simulink model "ASM_Traffic_MultiCore"  (R2026a)
settings: Solver=ode1  StartTime=SIM.tstart.v  StopTime=SIM.tend.v  FixedStep=SIM.StepSize.v
PostLoadFcn:
  | if any(exist('dsrtsu_mdlpostloadfcn', 'file') ~= 0), dsrtsu_mdlpostloadfcn('Execute', bdroot); end
  | try, asm_mdl_postloadfcn(bdroot, 'UpdateModel', 3600); catch, disp(lasterr); end,
InitFcn:
  | , if any(exist('rtifpga_mdlclblib', 'file') ~= 0), rtifpga_mdlclblib('Init', bdroot); end,
  | , if any(exist('dsmpb_private', 'file') ~= 0), dsmpb_private('dsmpb_mdlclblib', 'Init', bdroot); end,
model workspace (MAT data in the model file):
  asmReferencePath = [0 0.01 0.02 0.03 0.04 0.05 0.06 0.07 0.08 0.09 0.1 0.11 ... (350007 elements, 50001x7)]
  roadBounds : Simulink.Parameter (value not decoded)
  safetyAxes : Simulink.Parameter (value not decoded)
undefined symbols (not defined in the file): _to_, a0b2, ASM_BrakeHydraulics_DemoSystems, ASM_VehicleDynamics_DemoSystems, b98103fe8ad365046cd0, BrakeCircuit, controllerConfig, CPT, Crankshaft, DiscIntNeverNeededParam, dsmsi, FinalDriveAssembly, MDL, ModeSignals, mu, Pos_BrakePedal_Maneuver, rad, RefSignals, roadFamilyData, roadFamilyId, s_to_rpm, SIM, SoftECU, Suspension, Tire, Transmission
libraries: ASM_Traffic_lib x135, simulink x98, ASM_Utils_lib x77, ASM_VehicleDynamics_lib x70, ASM_Environment_lib x22, dsmpblib x20, dsmsilib x15, MDLD_Utils_lib x10, ASM_BrakeHydraulics_lib x3, sl_discontinuities x2
(part 55 of 65)

== system ASM_Traffic_MultiCore/VehicleDynamics/Plant/UserInterface/DISP_Plant/Positions/Angle_Pitch_Vehicle_CoorSys_E[deg] ==
  In1 : Inport
  Out1 : Outport  VectorParamsAs1DForOutWhenUnconnected=off
  wires:
  In1/1 -> Out1/1

== system ASM_Traffic_MultiCore/VehicleDynamics/Plant/UserInterface/DISP_Plant/Positions/Angle_Roll_Vehicle_CoorSys_E[deg] ==
  In1 : Inport
  Out1 : Outport  VectorParamsAs1DForOutWhenUnconnected=off
  wires:
  In1/1 -> Out1/1

== system ASM_Traffic_MultiCore/VehicleDynamics/Plant/UserInterface/DISP_Plant/Positions/Angle_Yaw_Vehicle_CoorSys_E[deg] ==
  In1 : Inport
  Out1 : Outport  VectorParamsAs1DForOutWhenUnconnected=off
  wires:
  In1/1 -> Out1/1

== system ASM_Traffic_MultiCore/VehicleDynamics/Plant/UserInterface/DISP_Plant/Positions/Pos_x_Vehicle_CoorSys_E[m] ==
  In1 : Inport
  Out1 : Outport  VectorParamsAs1DForOutWhenUnconnected=off
  wires:
  In1/1 -> Out1/1

== system ASM_Traffic_MultiCore/VehicleDynamics/Plant/UserInterface/DISP_Plant/Positions/Pos_y_Vehicle_CoorSys_E[m] ==
  In1 : Inport
  Out1 : Outport  VectorParamsAs1DForOutWhenUnconnected=off
  wires:
  In1/1 -> Out1/1

== system ASM_Traffic_MultiCore/VehicleDynamics/Plant/UserInterface/DISP_Plant/Positions/Pos_z_Vehicle_CoorSys_E[m] ==
  In1 : Inport
  Out1 : Outport  VectorParamsAs1DForOutWhenUnconnected=off
  wires:
  In1/1 -> Out1/1

== system ASM_Traffic_MultiCore/VehicleDynamics/Plant/UserInterface/DISP_Plant/Positions/s_Vehicle[m] ==
  In1 : Inport
  Out1 : Outport  VectorParamsAs1DForOutWhenUnconnected=off
  wires:
  In1/1 -> Out1/1

== system ASM_Traffic_MultiCore/VehicleDynamics/Plant/UserInterface/DISP_Plant/Sensor1/a_Angular_Sensor1_CoorSys_VH[x;y;z][rad|s2] ==
  In1 : Inport
  Out1 : Outport  VectorParamsAs1DForOutWhenUnconnected=off
  wires:
  In1/1 -> Out1/1

== system ASM_Traffic_MultiCore/VehicleDynamics/Plant/UserInterface/DISP_Plant/Sensor1/a_Angular_Sensor1_CoorSys_V[x;y;z][rad|s2] ==
  In1 : Inport
  Out1 : Outport  VectorParamsAs1DForOutWhenUnconnected=off
  wires:
  In1/1 -> Out1/1

== system ASM_Traffic_MultiCore/VehicleDynamics/Plant/UserInterface/DISP_Plant/Sensor1/a_Sensor1_CoorSys_VH[x;y;z][m|s2] ==
  In1 : Inport
  Out1 : Outport  VectorParamsAs1DForOutWhenUnconnected=off
  wires:
  In1/1 -> Out1/1

== system ASM_Traffic_MultiCore/VehicleDynamics/Plant/UserInterface/DISP_Plant/Sensor1/a_Sensor1_CoorSys_V[x;y;z][m|s2] ==
  In1 : Inport
  Out1 : Outport  VectorParamsAs1DForOutWhenUnconnected=off
  wires:
  In1/1 -> Out1/1

== system ASM_Traffic_MultiCore/VehicleDynamics/Plant/UserInterface/DISP_Plant/Sensor1/a_Total_Sensor1_CoorSys_VH[x;y;z][m|s2] ==
  In1 : Inport
  Out1 : Outport  VectorParamsAs1DForOutWhenUnconnected=off
  wires:
  In1/1 -> Out1/1

== system ASM_Traffic_MultiCore/VehicleDynamics/Plant/UserInterface/DISP_Plant/Sensor1/a_Total_Sensor1_CoorSys_V[x;y;z][m|s2] ==
  In1 : Inport
  Out1 : Outport  VectorParamsAs1DForOutWhenUnconnected=off
  wires:
  In1/1 -> Out1/1

== system ASM_Traffic_MultiCore/VehicleDynamics/Plant/UserInterface/DISP_Plant/Sensor1/v_Sensor1_CoorSys_VH[x;y;z][m|s] ==
  In1 : Inport
  Out1 : Outport  VectorParamsAs1DForOutWhenUnconnected=off
  wires:
  In1/1 -> Out1/1

== system ASM_Traffic_MultiCore/VehicleDynamics/Plant/UserInterface/DISP_Plant/Sensor1/v_Sensor1_CoorSys_V[x;y;z][m|s] ==
  In1 : Inport
  Out1 : Outport  VectorParamsAs1DForOutWhenUnconnected=off
  wires:
  In1/1 -> Out1/1

== system ASM_Traffic_MultiCore/VehicleDynamics/Plant/UserInterface/DISP_Plant/Sensor1/w_Sensor1_CoorSys_VH[x;y;z][rad|s] ==
  In1 : Inport
  Out1 : Outport  VectorParamsAs1DForOutWhenUnconnected=off
  wires:
  In1/1 -> Out1/1

== system ASM_Traffic_MultiCore/VehicleDynamics/Plant/UserInterface/DISP_Plant/Sensor1/w_Sensor1_CoorSys_V[x;y;z][rad|s] ==
  In1 : Inport
  Out1 : Outport  VectorParamsAs1DForOutWhenUnconnected=off
  wires:
  In1/1 -> Out1/1

== system ASM_Traffic_MultiCore/VehicleDynamics/Plant/UserInterface/DISP_Plant/Steering/Angle_SteeringGear[deg] ==
  In1 : Inport
  Out1 : Outport  VectorParamsAs1DForOutWhenUnconnected=off
  wires:
  In1/1 -> Out1/1

== system ASM_Traffic_MultiCore/VehicleDynamics/Plant/UserInterface/DISP_Plant/Steering/Angle_SteeringWheel[deg] ==
  In1 : Inport
  Out1 : Outport  VectorParamsAs1DForOutWhenUnconnected=off
  wires:
  In1/1 -> Out1/1

== system ASM_Traffic_MultiCore/VehicleDynamics/Plant/UserInterface/DISP_Plant/Steering/Displ_Steering[m] ==
  In1 : Inport
  Out1 : Outport  VectorParamsAs1DForOutWhenUnconnected=off
  wires:
  In1/1 -> Out1/1

== system ASM_Traffic_MultiCore/VehicleDynamics/Plant/UserInterface/DISP_Plant/Steering/Trq_PowerSteering[Nm] ==
  In1 : Inport
  Out1 : Outport  VectorParamsAs1DForOutWhenUnconnected=off
  wires:
  In1/1 -> Out1/1

== system ASM_Traffic_MultiCore/VehicleDynamics/Plant/UserInterface/DISP_Plant/Steering/Trq_Steering[Nm] ==
  In1 : Inport
  Out1 : Outport  VectorParamsAs1DForOutWhenUnconnected=off
  wires:
  In1/1 -> Out1/1

== system ASM_Traffic_MultiCore/VehicleDynamics/Plant/UserInterface/DISP_Plant/Steering/i_Steering_Mean[] ==
  In1 : Inport
  Out1 : Outport  VectorParamsAs1DForOutWhenUnconnected=off
  wires:
  In1/1 -> Out1/1

== system ASM_Traffic_MultiCore/VehicleDynamics/Plant/UserInterface/DISP_Plant/Suspension/Angle_Alpha_FL_Wheel[deg] ==
  In1 : Inport
  Out1 : Outport  VectorParamsAs1DForOutWhenUnconnected=off
  wires:
  In1/1 -> Out1/1

== system ASM_Traffic_MultiCore/VehicleDynamics/Plant/UserInterface/DISP_Plant/Suspension/Angle_Alpha_FR_Wheel[deg] ==
  In1 : Inport
  Out1 : Outport  VectorParamsAs1DForOutWhenUnconnected=off
  wires:
  In1/1 -> Out1/1

== system ASM_Traffic_MultiCore/VehicleDynamics/Plant/UserInterface/DISP_Plant/Suspension/Angle_Alpha_RL_Wheel[deg] ==
  In1 : Inport
  Out1 : Outport  VectorParamsAs1DForOutWhenUnconnected=off
  wires:
  In1/1 -> Out1/1

== system ASM_Traffic_MultiCore/VehicleDynamics/Plant/UserInterface/DISP_Plant/Suspension/Angle_Alpha_RR_Wheel[deg] ==
  In1 : Inport
  Out1 : Outport  VectorParamsAs1DForOutWhenUnconnected=off
  wires:
  In1/1 -> Out1/1

== system ASM_Traffic_MultiCore/VehicleDynamics/Plant/UserInterface/DISP_Plant/Suspension/Angle_Beta_FL_Wheel[deg] ==
  In1 : Inport
  Out1 : Outport  VectorParamsAs1DForOutWhenUnconnected=off
  wires:
  In1/1 -> Out1/1

== system ASM_Traffic_MultiCore/VehicleDynamics/Plant/UserInterface/DISP_Plant/Suspension/Angle_Beta_FR_Wheel[deg] ==
  In1 : Inport
  Out1 : Outport  VectorParamsAs1DForOutWhenUnconnected=off
  wires:
  In1/1 -> Out1/1

== system ASM_Traffic_MultiCore/VehicleDynamics/Plant/UserInterface/DISP_Plant/Suspension/Angle_Beta_RL_Wheel[deg] ==
  In1 : Inport
  Out1 : Outport  VectorParamsAs1DForOutWhenUnconnected=off
  wires:
  In1/1 -> Out1/1

== system ASM_Traffic_MultiCore/VehicleDynamics/Plant/UserInterface/DISP_Plant/Suspension/Angle_Beta_RR_Wheel[deg] ==
  In1 : Inport
  Out1 : Outport  VectorParamsAs1DForOutWhenUnconnected=off
  wires:
  In1/1 -> Out1/1

== system ASM_Traffic_MultiCore/VehicleDynamics/Plant/UserInterface/DISP_Plant/Suspension/Angle_FL_Wheel[Alpha;Beta;Gamma][deg] ==
  In1 : Inport
  Out1 : Outport  VectorParamsAs1DForOutWhenUnconnected=off
  wires:
  In1/1 -> Out1/1

== system ASM_Traffic_MultiCore/VehicleDynamics/Plant/UserInterface/DISP_Plant/Suspension/Angle_FRWheel[Alpha;Beta;Gamma][deg] ==
  In1 : Inport
  Out1 : Outport  VectorParamsAs1DForOutWhenUnconnected=off
  wires:
  In1/1 -> Out1/1

== system ASM_Traffic_MultiCore/VehicleDynamics/Plant/UserInterface/DISP_Plant/Suspension/Angle_Gamma_FL_Wheel[deg] ==
  In1 : Inport
  Out1 : Outport  VectorParamsAs1DForOutWhenUnconnected=off
  wires:
  In1/1 -> Out1/1

== system ASM_Traffic_MultiCore/VehicleDynamics/Plant/UserInterface/DISP_Plant/Suspension/Angle_Gamma_FR_Wheel[deg] ==
  In1 : Inport
  Out1 : Outport  VectorParamsAs1DForOutWhenUnconnected=off
  wires:
  In1/1 -> Out1/1

== system ASM_Traffic_MultiCore/VehicleDynamics/Plant/UserInterface/DISP_Plant/Suspension/Angle_Gamma_RL_Wheel[deg] ==
  In1 : Inport
  Out1 : Outport  VectorParamsAs1DForOutWhenUnconnected=off
  wires:
  In1/1 -> Out1/1

== system ASM_Traffic_MultiCore/VehicleDynamics/Plant/UserInterface/DISP_Plant/Suspension/Angle_Gamma_RR_Wheel[deg] ==
  In1 : Inport
  Out1 : Outport  VectorParamsAs1DForOutWhenUnconnected=off
  wires:
  In1/1 -> Out1/1

== system ASM_Traffic_MultiCore/VehicleDynamics/Plant/UserInterface/DISP_Plant/Suspension/Angle_RL_Wheel[Alpha;Beta;Gamma][deg] ==
  In1 : Inport
  Out1 : Outport  VectorParamsAs1DForOutWhenUnconnected=off
  wires:
  In1/1 -> Out1/1

== system ASM_Traffic_MultiCore/VehicleDynamics/Plant/UserInterface/DISP_Plant/Suspension/Angle_RR_Wheel[Alpha;Beta;Gamma][deg] ==
  In1 : Inport
  Out1 : Outport  VectorParamsAs1DForOutWhenUnconnected=off
  wires:
  In1/1 -> Out1/1

== system ASM_Traffic_MultiCore/VehicleDynamics/Plant/UserInterface/DISP_Plant/Suspension/Displ_Damper_FL[m] ==
  In1 : Inport
  Out1 : Outport  VectorParamsAs1DForOutWhenUnconnected=off
  wires:
  In1/1 -> Out1/1

== system ASM_Traffic_MultiCore/VehicleDynamics/Plant/UserInterface/DISP_Plant/Suspension/Displ_Damper_FL_dt[m|s] ==
  In1 : Inport
  Out1 : Outport  VectorParamsAs1DForOutWhenUnconnected=off
  wires:
  In1/1 -> Out1/1

== system ASM_Traffic_MultiCore/VehicleDynamics/Plant/UserInterface/DISP_Plant/Suspension/Displ_Damper_FR[m] ==
  In1 : Inport
  Out1 : Outport  VectorParamsAs1DForOutWhenUnconnected=off
  wires:
  In1/1 -> Out1/1

== system ASM_Traffic_MultiCore/VehicleDynamics/Plant/UserInterface/DISP_Plant/Suspension/Displ_Damper_FR_dt[m|s] ==
  In1 : Inport
  Out1 : Outport  VectorParamsAs1DForOutWhenUnconnected=off
  wires:
  In1/1 -> Out1/1

== system ASM_Traffic_MultiCore/VehicleDynamics/Plant/UserInterface/DISP_Plant/Suspension/Displ_Damper_RL[m] ==
  In1 : Inport
  Out1 : Outport  VectorParamsAs1DForOutWhenUnconnected=off
  wires:
  In1/1 -> Out1/1

== system ASM_Traffic_MultiCore/VehicleDynamics/Plant/UserInterface/DISP_Plant/Suspension/Displ_Damper_RL_dt[m|s] ==
  In1 : Inport
  Out1 : Outport  VectorParamsAs1DForOutWhenUnconnected=off
  wires:
  In1/1 -> Out1/1

== system ASM_Traffic_MultiCore/VehicleDynamics/Plant/UserInterface/DISP_Plant/Suspension/Displ_Damper_RR[m] ==
  In1 : Inport
  Out1 : Outport  VectorParamsAs1DForOutWhenUnconnected=off
  wires:
  In1/1 -> Out1/1

== system ASM_Traffic_MultiCore/VehicleDynamics/Plant/UserInterface/DISP_Plant/Suspension/Displ_Damper_RR_dt[m|s] ==
  In1 : Inport
  Out1 : Outport  VectorParamsAs1DForOutWhenUnconnected=off
  wires:
  In1/1 -> Out1/1

== system ASM_Traffic_MultiCore/VehicleDynamics/Plant/UserInterface/DISP_Plant/Suspension/Displ_Spring_FL[m] ==
  In1 : Inport
  Out1 : Outport  VectorParamsAs1DForOutWhenUnconnected=off
  wires:
  In1/1 -> Out1/1

== system ASM_Traffic_MultiCore/VehicleDynamics/Plant/UserInterface/DISP_Plant/Suspension/Displ_Spring_FRm] ==
  In1 : Inport
  Out1 : Outport  VectorParamsAs1DForOutWhenUnconnected=off
  wires:
  In1/1 -> Out1/1

== system ASM_Traffic_MultiCore/VehicleDynamics/Plant/UserInterface/DISP_Plant/Suspension/Displ_Spring_RL[m] ==
  In1 : Inport
  Out1 : Outport  VectorParamsAs1DForOutWhenUnconnected=off
  wires:
  In1/1 -> Out1/1

== system ASM_Traffic_MultiCore/VehicleDynamics/Plant/UserInterface/DISP_Plant/Suspension/Displ_Spring_RR[m] ==
  In1 : Inport
  Out1 : Outport  VectorParamsAs1DForOutWhenUnconnected=off
  wires:
  In1/1 -> Out1/1

== system ASM_Traffic_MultiCore/VehicleDynamics/Plant/UserInterface/DISP_Plant/Suspension/Displ_Stabilizer_Front[m] ==
  In1 : Inport
  Out1 : Outport  VectorParamsAs1DForOutWhenUnconnected=off
  wires:
  In1/1 -> Out1/1

== system ASM_Traffic_MultiCore/VehicleDynamics/Plant/UserInterface/DISP_Plant/Suspension/Displ_Stabilizer_Rear[m] ==
  In1 : Inport
  Out1 : Outport  VectorParamsAs1DForOutWhenUnconnected=off
  wires:
  In1/1 -> Out1/1

== system ASM_Traffic_MultiCore/VehicleDynamics/Plant/UserInterface/DISP_Plant/Suspension/F_FL_Damper[N] ==
  In1 : Inport
  Out1 : Outport  VectorParamsAs1DForOutWhenUnconnected=off
  wires:
  In1/1 -> Out1/1

== system ASM_Traffic_MultiCore/VehicleDynamics/Plant/UserInterface/DISP_Plant/Suspension/F_FL_Spring[N] ==
  In1 : Inport
  Out1 : Outport  VectorParamsAs1DForOutWhenUnconnected=off
  wires:
  In1/1 -> Out1/1

== system ASM_Traffic_MultiCore/VehicleDynamics/Plant/UserInterface/DISP_Plant/Suspension/F_FR_Damper[N] ==
  In1 : Inport
  Out1 : Outport  VectorParamsAs1DForOutWhenUnconnected=off
  wires:
  In1/1 -> Out1/1

== system ASM_Traffic_MultiCore/VehicleDynamics/Plant/UserInterface/DISP_Plant/Suspension/F_FR_Spring[N] ==
  In1 : Inport
  Out1 : Outport  VectorParamsAs1DForOutWhenUnconnected=off
  wires:
  In1/1 -> Out1/1

== system ASM_Traffic_MultiCore/VehicleDynamics/Plant/UserInterface/DISP_Plant/Suspension/F_RL_Damper[N] ==
  In1 : Inport
  Out1 : Outport  VectorParamsAs1DForOutWhenUnconnected=off
  wires:
  In1/1 -> Out1/1

== system ASM_Traffic_MultiCore/VehicleDynamics/Plant/UserInterface/DISP_Plant/Suspension/F_RL_Spring[N] ==
  In1 : Inport
  Out1 : Outport  VectorParamsAs1DForOutWhenUnconnected=off
  wires:
  In1/1 -> Out1/1

== system ASM_Traffic_MultiCore/VehicleDynamics/Plant/UserInterface/DISP_Plant/Suspension/F_RR_Damper[N] ==
  In1 : Inport
  Out1 : Outport  VectorParamsAs1DForOutWhenUnconnected=off
  wires:
  In1/1 -> Out1/1

== system ASM_Traffic_MultiCore/VehicleDynamics/Plant/UserInterface/DISP_Plant/Suspension/F_RR_Spring[N] ==
  In1 : Inport
  Out1 : Outport  VectorParamsAs1DForOutWhenUnconnected=off
  wires:
  In1/1 -> Out1/1

== system ASM_Traffic_MultiCore/VehicleDynamics/Plant/UserInterface/DISP_Plant/Suspension/F_Stabilizer_Front[N] ==
  In1 : Inport
  Out1 : Outport  VectorParamsAs1DForOutWhenUnconnected=off
  wires:
  In1/1 -> Out1/1

== system ASM_Traffic_MultiCore/VehicleDynamics/Plant/UserInterface/DISP_Plant/Suspension/F_Stabilizer_Rear[N] ==
  In1 : Inport
  Out1 : Outport  VectorParamsAs1DForOutWhenUnconnected=off
  wires:
  In1/1 -> Out1/1

== system ASM_Traffic_MultiCore/VehicleDynamics/Plant/UserInterface/DISP_Plant/Suspension/Pos_FL_Wheel[x;y;z][m] ==
  In1 : Inport
  Out1 : Outport  VectorParamsAs1DForOutWhenUnconnected=off
  wires:
  In1/1 -> Out1/1

== system ASM_Traffic_MultiCore/VehicleDynamics/Plant/UserInterface/DISP_Plant/Suspension/Pos_FR_Wheel[x;y;z][m] ==
  In1 : Inport
  Out1 : Outport  VectorParamsAs1DForOutWhenUnconnected=off
  wires:
  In1/1 -> Out1/1

== system ASM_Traffic_MultiCore/VehicleDynamics/Plant/UserInterface/DISP_Plant/Suspension/Pos_RL_Wheel[x;y;z][m] ==
  In1 : Inport
  Out1 : Outport  VectorParamsAs1DForOutWhenUnconnected=off
  wires:
  In1/1 -> Out1/1

== system ASM_Traffic_MultiCore/VehicleDynamics/Plant/UserInterface/DISP_Plant/Suspension/Pos_RR_Wheel[x;y;z][m] ==
  In1 : Inport
  Out1 : Outport  VectorParamsAs1DForOutWhenUnconnected=off
  wires:
  In1/1 -> Out1/1

== system ASM_Traffic_MultiCore/VehicleDynamics/Plant/UserInterface/DISP_Plant/Tire/F_x_Dyn_FL_Tire_CoorSys_CP[N] ==
  In1 : Inport
  Out1 : Outport  VectorParamsAs1DForOutWhenUnconnected=off
  wires:
  In1/1 -> Out1/1

== system ASM_Traffic_MultiCore/VehicleDynamics/Plant/UserInterface/DISP_Plant/Tire/F_x_Dyn_FR_Tire_CoorSys_CP[N] ==
  In1 : Inport
  Out1 : Outport  VectorParamsAs1DForOutWhenUnconnected=off
  wires:
  In1/1 -> Out1/1

== system ASM_Traffic_MultiCore/VehicleDynamics/Plant/UserInterface/DISP_Plant/Tire/F_x_Dyn_RL_Tire_CoorSys_CP[N] ==
  In1 : Inport
  Out1 : Outport  VectorParamsAs1DForOutWhenUnconnected=off
  wires:
  In1/1 -> Out1/1

== system ASM_Traffic_MultiCore/VehicleDynamics/Plant/UserInterface/DISP_Plant/Tire/F_x_Dyn_RR_Tire_CoorSys_CP[N] ==
  In1 : Inport
  Out1 : Outport  VectorParamsAs1DForOutWhenUnconnected=off
  wires:
  In1/1 -> Out1/1

== system ASM_Traffic_MultiCore/VehicleDynamics/Plant/UserInterface/DISP_Plant/Tire/F_y_Dyn_FL_Tire_CoorSys_CP[N] ==
  In1 : Inport
  Out1 : Outport  VectorParamsAs1DForOutWhenUnconnected=off
  wires:
  In1/1 -> Out1/1

== system ASM_Traffic_MultiCore/VehicleDynamics/Plant/UserInterface/DISP_Plant/Tire/F_y_Dyn_FR_Tire_CoorSys_CP[N] ==
  In1 : Inport
  Out1 : Outport  VectorParamsAs1DForOutWhenUnconnected=off
  wires:
  In1/1 -> Out1/1

== system ASM_Traffic_MultiCore/VehicleDynamics/Plant/UserInterface/DISP_Plant/Tire/F_y_Dyn_RL_Tire_CoorSys_CP[N] ==
  In1 : Inport
  Out1 : Outport  VectorParamsAs1DForOutWhenUnconnected=off
  wires:
  In1/1 -> Out1/1

== system ASM_Traffic_MultiCore/VehicleDynamics/Plant/UserInterface/DISP_Plant/Tire/F_y_Dyn_RR_Tire_CoorSys_CP[N] ==
  In1 : Inport
  Out1 : Outport  VectorParamsAs1DForOutWhenUnconnected=off
  wires:
  In1/1 -> Out1/1

== system ASM_Traffic_MultiCore/VehicleDynamics/Plant/UserInterface/DISP_Plant/Tire/F_z_Dyn_FL_Tire_CoorSys_CP[N] ==
  In1 : Inport
  Out1 : Outport  VectorParamsAs1DForOutWhenUnconnected=off
  wires:
  In1/1 -> Out1/1

== system ASM_Traffic_MultiCore/VehicleDynamics/Plant/UserInterface/DISP_Plant/Tire/F_z_Dyn_FR_Tire_CoorSys_CP[N] ==
  In1 : Inport
  Out1 : Outport  VectorParamsAs1DForOutWhenUnconnected=off
  wires:
  In1/1 -> Out1/1

== system ASM_Traffic_MultiCore/VehicleDynamics/Plant/UserInterface/DISP_Plant/Tire/F_z_Dyn_RL_Tire_CoorSys_CP[N] ==
  In1 : Inport
  Out1 : Outport  VectorParamsAs1DForOutWhenUnconnected=off
  wires:
  In1/1 -> Out1/1

== system ASM_Traffic_MultiCore/VehicleDynamics/Plant/UserInterface/DISP_Plant/Tire/F_z_Dyn_RR_Tire_CoorSys_CP[N] ==
  In1 : Inport
  Out1 : Outport  VectorParamsAs1DForOutWhenUnconnected=off
  wires:
  In1/1 -> Out1/1

== system ASM_Traffic_MultiCore/VehicleDynamics/Plant/UserInterface/DISP_Plant/Tire/Slip_x_FL[] ==
  In1 : Inport
  Out1 : Outport  VectorParamsAs1DForOutWhenUnconnected=off
  wires:
  In1/1 -> Out1/1

== system ASM_Traffic_MultiCore/VehicleDynamics/Plant/UserInterface/DISP_Plant/Tire/Slip_x_FR[] ==
  In1 : Inport
  Out1 : Outport  VectorParamsAs1DForOutWhenUnconnected=off
  wires:
  In1/1 -> Out1/1

== system ASM_Traffic_MultiCore/VehicleDynamics/Plant/UserInterface/DISP_Plant/Tire/Slip_x_RL[] ==
  In1 : Inport
  Out1 : Outport  VectorParamsAs1DForOutWhenUnconnected=off
  wires:
  In1/1 -> Out1/1

== system ASM_Traffic_MultiCore/VehicleDynamics/Plant/UserInterface/DISP_Plant/Tire/Slip_x_RR[] ==
  In1 : Inport
  Out1 : Outport  VectorParamsAs1DForOutWhenUnconnected=off
  wires:
  In1/1 -> Out1/1

== system ASM_Traffic_MultiCore/VehicleDynamics/Plant/UserInterface/DISP_Plant/Tire/Slip_y_FL[] ==
  In1 : Inport
  Out1 : Outport  VectorParamsAs1DForOutWhenUnconnected=off
  wires:
  In1/1 -> Out1/1

== system ASM_Traffic_MultiCore/VehicleDynamics/Plant/UserInterface/DISP_Plant/Tire/Slip_y_FR[] ==
  In1 : Inport
  Out1 : Outport  VectorParamsAs1DForOutWhenUnconnected=off
  wires:
  In1/1 -> Out1/1

== system ASM_Traffic_MultiCore/VehicleDynamics/Plant/UserInterface/DISP_Plant/Tire/Slip_y_RL[] ==
  In1 : Inport
  Out1 : Outport  VectorParamsAs1DForOutWhenUnconnected=off
  wires:
  In1/1 -> Out1/1

== system ASM_Traffic_MultiCore/VehicleDynamics/Plant/UserInterface/DISP_Plant/Tire/Slip_y_RR[] ==
  In1 : Inport
  Out1 : Outport  VectorParamsAs1DForOutWhenUnconnected=off
  wires:
  In1/1 -> Out1/1

== system ASM_Traffic_MultiCore/VehicleDynamics/Plant/UserInterface/DISP_Plant/Tire/Trq_x_FL_CoorSys_CP[Nm] ==
  In1 : Inport
  Out1 : Outport  VectorParamsAs1DForOutWhenUnconnected=off
  wires:
  In1/1 -> Out1/1

== system ASM_Traffic_MultiCore/VehicleDynamics/Plant/UserInterface/DISP_Plant/Tire/Trq_x_FR_CoorSys_CP[Nm] ==
  In1 : Inport
  Out1 : Outport  VectorParamsAs1DForOutWhenUnconnected=off
  wires:
  In1/1 -> Out1/1

== system ASM_Traffic_MultiCore/VehicleDynamics/Plant/UserInterface/DISP_Plant/Tire/Trq_x_RL_CoorSys_CP[Nm] ==
  In1 : Inport
  Out1 : Outport  VectorParamsAs1DForOutWhenUnconnected=off
  wires:
  In1/1 -> Out1/1

== system ASM_Traffic_MultiCore/VehicleDynamics/Plant/UserInterface/DISP_Plant/Tire/Trq_x_RR_CoorSys_CP[Nm] ==
  In1 : Inport
  Out1 : Outport  VectorParamsAs1DForOutWhenUnconnected=off
  wires:
  In1/1 -> Out1/1

== system ASM_Traffic_MultiCore/VehicleDynamics/Plant/UserInterface/DISP_Plant/Tire/Trq_y_FL_CoorSys_W[Nm] ==
  In1 : Inport
  Out1 : Outport  VectorParamsAs1DForOutWhenUnconnected=off
  wires:
  In1/1 -> Out1/1

== system ASM_Traffic_MultiCore/VehicleDynamics/Plant/UserInterface/DISP_Plant/Tire/Trq_y_FR_CoorSys_W[Nm] ==
  In1 : Inport
  Out1 : Outport  VectorParamsAs1DForOutWhenUnconnected=off
  wires:
  In1/1 -> Out1/1

== system ASM_Traffic_MultiCore/VehicleDynamics/Plant/UserInterface/DISP_Plant/Tire/Trq_y_RL_CoorSys_W[Nm] ==
  In1 : Inport
  Out1 : Outport  VectorParamsAs1DForOutWhenUnconnected=off
  wires:
  In1/1 -> Out1/1

== system ASM_Traffic_MultiCore/VehicleDynamics/Plant/UserInterface/DISP_Plant/Tire/Trq_y_RR_CoorSys_W[Nm] ==
  In1 : Inport
  Out1 : Outport  VectorParamsAs1DForOutWhenUnconnected=off
  wires:
  In1/1 -> Out1/1

== system ASM_Traffic_MultiCore/VehicleDynamics/Plant/UserInterface/DISP_Plant/Tire/Trq_z_FL_CoorSys_CP[Nm] ==
  In1 : Inport
  Out1 : Outport  VectorParamsAs1DForOutWhenUnconnected=off
  wires:
  In1/1 -> Out1/1

== system ASM_Traffic_MultiCore/VehicleDynamics/Plant/UserInterface/DISP_Plant/Tire/Trq_z_FR_CoorSys_CP[Nm] ==
  In1 : Inport
  Out1 : Outport  VectorParamsAs1DForOutWhenUnconnected=off
  wires:
  In1/1 -> Out1/1

== system ASM_Traffic_MultiCore/VehicleDynamics/Plant/UserInterface/DISP_Plant/Tire/Trq_z_RL_CoorSys_CP[Nm] ==
  In1 : Inport
  Out1 : Outport  VectorParamsAs1DForOutWhenUnconnected=off
  wires:
  In1/1 -> Out1/1

== system ASM_Traffic_MultiCore/VehicleDynamics/Plant/UserInterface/DISP_Plant/Tire/Trq_z_RR_CoorSys_CP[Nm] ==
  In1 : Inport
  Out1 : Outport  VectorParamsAs1DForOutWhenUnconnected=off
  wires:
  In1/1 -> Out1/1

== system ASM_Traffic_MultiCore/VehicleDynamics/Plant/UserInterface/DISP_Plant/Tire/r_Dyn_FL_Tire[m] ==
  In1 : Inport
  Out1 : Outport  VectorParamsAs1DForOutWhenUnconnected=off
  wires:
  In1/1 -> Out1/1

== system ASM_Traffic_MultiCore/VehicleDynamics/Plant/UserInterface/DISP_Plant/Tire/r_Dyn_FR_Tire[m] ==
  In1 : Inport
  Out1 : Outport  VectorParamsAs1DForOutWhenUnconnected=off
  wires:
  In1/1 -> Out1/1

== system ASM_Traffic_MultiCore/VehicleDynamics/Plant/UserInterface/DISP_Plant/Tire/r_Dyn_RL_Tire[m] ==
  In1 : Inport
  Out1 : Outport  VectorParamsAs1DForOutWhenUnconnected=off
  wires:
  In1/1 -> Out1/1

== system ASM_Traffic_MultiCore/VehicleDynamics/Plant/UserInterface/DISP_Plant/Tire/r_Dyn_RR_Tire[m] ==
  In1 : Inport
  Out1 : Outport  VectorParamsAs1DForOutWhenUnconnected=off
  wires:
  In1/1 -> Out1/1

== system ASM_Traffic_MultiCore/VehicleDynamics/Plant/UserInterface/DISP_Plant/Tire/v_Circumf_Dyn_FL_Wheel[km|h] ==
  In1 : Inport
  Out1 : Outport  VectorParamsAs1DForOutWhenUnconnected=off
  wires:
  In1/1 -> Out1/1

== system ASM_Traffic_MultiCore/VehicleDynamics/Plant/UserInterface/DISP_Plant/Tire/v_Circumf_Dyn_FR_Wheel[km|h] ==
  In1 : Inport
  Out1 : Outport  VectorParamsAs1DForOutWhenUnconnected=off
  wires:
  In1/1 -> Out1/1

== system ASM_Traffic_MultiCore/VehicleDynamics/Plant/UserInterface/DISP_Plant/Tire/v_Circumf_Dyn_RL_Wheel[km|h] ==
  In1 : Inport
  Out1 : Outport  VectorParamsAs1DForOutWhenUnconnected=off
  wires:
  In1/1 -> Out1/1

== system ASM_Traffic_MultiCore/VehicleDynamics/Plant/UserInterface/DISP_Plant/Tire/v_Circumf_Dyn_RR_Wheel[km|h] ==
  In1 : Inport
  Out1 : Outport  VectorParamsAs1DForOutWhenUnconnected=off
  wires:
  In1/1 -> Out1/1

== system ASM_Traffic_MultiCore/VehicleDynamics/Plant/UserInterface/DISP_Plant/Velocities/Angle_SideSlip_Vehicle[deg] ==
  In1 : Inport
  Out1 : Outport  VectorParamsAs1DForOutWhenUnconnected=off
  wires:
  In1/1 -> Out1/1

== system ASM_Traffic_MultiCore/VehicleDynamics/Plant/UserInterface/DISP_Plant/Velocities/PitchRate_Vehicle_CoG[deg|s] ==
  In1 : Inport
  Out1 : Outport  VectorParamsAs1DForOutWhenUnconnected=off
  wires:
  In1/1 -> Out1/1

== system ASM_Traffic_MultiCore/VehicleDynamics/Plant/UserInterface/DISP_Plant/Velocities/RollRate_Vehicle_CoG[deg|s] ==
  In1 : Inport
  Out1 : Outport  VectorParamsAs1DForOutWhenUnconnected=off
  wires:
  In1/1 -> Out1/1

== system ASM_Traffic_MultiCore/VehicleDynamics/Plant/UserInterface/DISP_Plant/Velocities/YawRate_Vehicle_CoG[deg|s] ==
  In1 : Inport
  Out1 : Outport  VectorParamsAs1DForOutWhenUnconnected=off
  wires:
  In1/1 -> Out1/1

== system ASM_Traffic_MultiCore/VehicleDynamics/Plant/UserInterface/DISP_Plant/Velocities/v_x_Vehicle_CoG[km|h] ==
  In1 : Inport
  Out1 : Outport  VectorParamsAs1DForOutWhenUnconnected=off
  wires:
  In1/1 -> Out1/1

== system ASM_Traffic_MultiCore/VehicleDynamics/Plant/UserInterface/DISP_Plant/Velocities/v_y_Vehicle_CoG[km|h] ==
  In1 : Inport
  Out1 : Outport  VectorParamsAs1DForOutWhenUnconnected=off
  wires:
  In1/1 -> Out1/1

== system ASM_Traffic_MultiCore/VehicleDynamics/Plant/UserInterface/DISP_Plant/Velocities/v_z_Vehicle_CoG[km|h] ==
  In1 : Inport
  Out1 : Outport  VectorParamsAs1DForOutWhenUnconnected=off
  wires:
  In1/1 -> Out1/1

== system ASM_Traffic_MultiCore/VehicleDynamics/Plant/UserInterface/DISP_Plant/WheelSpeeds/omega_FL_Wheel[rad|s] ==
  In1 : Inport
  Out1 : Outport  VectorParamsAs1DForOutWhenUnconnected=off
  wires:
  In1/1 -> Out1/1

== system ASM_Traffic_MultiCore/VehicleDynamics/Plant/UserInterface/DISP_Plant/WheelSpeeds/omega_FR_Wheel[rad|s] ==
  In1 : Inport
  Out1 : Outport  VectorParamsAs1DForOutWhenUnconnected=off
  wires:
  In1/1 -> Out1/1

== system ASM_Traffic_MultiCore/VehicleDynamics/Plant/UserInterface/DISP_Plant/WheelSpeeds/omega_RL_Wheel[rad|s] ==
  In1 : Inport
  Out1 : Outport  VectorParamsAs1DForOutWhenUnconnected=off
  wires:
  In1/1 -> Out1/1

== system ASM_Traffic_MultiCore/VehicleDynamics/Plant/UserInterface/DISP_Plant/WheelSpeeds/omega_RR_Wheel[rad|s] ==
  In1 : Inport
  Out1 : Outport  VectorParamsAs1DForOutWhenUnconnected=off
  wires:
  In1/1 -> Out1/1

== system ASM_Traffic_MultiCore/VehicleDynamics/Plant/VehicleDynamics/Brake/BRAKE_HYDRAULICS/ASMSignalCollector ==
  BusCreator : BusCreator  Inputs=2
  Const_BrakeHydraulicsModel[] : Constant  Value=2
      settings: AttributesFormatString=2 - Basic
  ASMSignalBus : Outport  VectorParamsAs1DForOutWhenUnconnected=off
  wires:
  BusCreator/1 -> ASMSignalBus/1  "BrakeHydraulics"
  Const_BrakeHydraulicsModel[]/1 -> BusCreator/2  "BrakeHydraulicsModel[]"
  [TAG_DISP_BrkHyd_BrakingCircuitBasic] -> BusCreator/1

== system ASM_Traffic_MultiCore/VehicleDynamics/Plant/VehicleDynamics/Suspension/SuspensionFront/ASMSignalCollector ==
  BusCreator1 : BusCreator  Inputs=4
  Terminator_1 : Terminator
  Terminator_2 : Terminator
  SuspensionFront : Outport  VectorParamsAs1DForOutWhenUnconnected=off
  wires:
  [ASMBUS_SuspensionKinematicsFront] -> BusCreator1/1  "SuspensionKinematicsFront"
  BusCreator1/1 -> SuspensionFront/1  "SuspensionFront"
  [ASMBUS_SuspensionForcesKinematicsFront] -> Terminator_1/1
  [ASMBUS_WheelRelativeVelocityFront] -> Terminator_2/1
  [ASMBUS_WheelRelativePositionFront] -> BusCreator1/4
  [ASMBUS_SuspensionComplianceFront] -> BusCreator1/2
  [ASMBUS_SuspensionForcesFront] -> BusCreator1/3

== system ASM_Traffic_MultiCore/VehicleDynamics/Plant/VehicleDynamics/Suspension/SuspensionFront/SusKin_Front ==
  Displ_SteeringRod[Left;Right][m] : Inport
  Displ_SteeringRod_dt[Left;Right][m|s] : Inport  Port=2
  Displ_z_Wheel[Left;Right][m] : Inport  Port=3
  Displ_z_dt_Wheel[Left;Right][m|s] : Inport  Port=4
  WheelPos_Offset[x;y;z][m] : Inport  Port=5
  Sw_Rotation[1Cardan|2ToeCamberSideView] : Inport  Port=6
  SUSKIN_SYM_FRONT : ASM_VehicleDynamics_lib/VehicleDynamics/Suspension/Base/SUSKIN_SYM  Tag=ASM_SUBCOMPONENT  Const_Pos_LeftWheel=MDL.VehicleDynamics.Suspension.Symmetric.Front.Const_Pos_LeftWheel  Map_Displ_x_LeftWheel_q1q2=MDL.VehicleDynamics.Suspension.Symmetric.Front.Map_Displ_x_LeftWheel_q1q2  Map_Displ_x_LeftWheel_q3=MDL.VehicleDynamics.Suspension.Symmetric.Front.Map_Displ_x_LeftWheel_q3  Map_Displ_y_LeftWheel_q1q2=MDL.VehicleDynamics.Suspension.Symmetric.Front.Map_Displ_y_LeftWheel_q1q2  Map_Displ_y_LeftWheel_q3=MDL.VehicleDynamics.Suspension.Symmetric.Front.Map_Displ_y_LeftWheel_q3  Map_Angle_Alpha_LeftWheel_q1q2=MDL.VehicleDynamics.Suspension.Symmetric.Front.Map_Angle_AlphaCamber_LeftWheel_q1q2  Map_Angle_Alpha_LeftWheel_q3=MDL.VehicleDynamics.Suspension.Symmetric.Front.Map_Angle_AlphaCamber_LeftWheel_q3  Map_Angle_Beta_LeftWheel_q1q2=MDL.VehicleDynamics.Suspension.Symmetric.Front.Map_Angle_BetaSideView_LeftWheel_q1q2  Map_Angle_Beta_LeftWheel_q3=MDL.VehicleDynamics.Suspension.Symmetric.Front.Map_Angle_BetaSideView_LeftWheel_q3  Map_Angle_Gamma_LeftWheel_q1q2=MDL.VehicleDynamics.Suspension.Symmetric.Front.Map_Angle_GammaToe_LeftWheel_q1q2  Map_Angle_Gamma_LeftWheel_q3=MDL.VehicleDynamics.Suspension.Symmetric.Front.Map_Angle_GammaToe_LeftWheel_q3  Map_Displ_Spring_Left_q1q2=MDL.VehicleDynamics.Suspension.Symmetric.Front.Map_Displ_Spring_Left_q1q2  Map_Displ_Spring_Left_q3=MDL.VehicleDynamics.Suspension.Symmetric.Front.Map_Displ_Spring_Left_q3  Map_Displ_Damper_Left_q1q2=MDL.VehicleDynamics.Suspension.Symmetric.Front.Map_Displ_Damper_Left_q1q2  Map_Displ_Damper_Left_q3=MDL.VehicleDynamics.Suspension.Symmetric.Front.Map_Displ_Damper_Left_q3  Map_Displ_Stabi_Left_q1q2=MDL.VehicleDynamics.Suspension.Symmetric.Front.Map_Displ_Stabilizer_Left_q1q2  Map_Displ_Stabi_Left_q3=MDL.VehicleDynamics.Suspension.Symmetric.Front.Map_Displ_Stabilizer_Left_q3  ASMProperties=struct('Name','SUSKIN_SYM','Version','2.0','Library','ASM_VehicleDynamics_lib')  ASMInstanceName=suskin_sym_front  ASMInstanceID=1
      settings: AttributesFormatString=Instance Name: %<ASMInstanceName>\nInstance ID: %<ASMInstanceID>
  Terminator : Terminator
  ASMSignalBus : Outport  VectorParamsAs1DForOutWhenUnconnected=off
  Pos_Left_Wheel_dq[qL;qR][x;y;z][] : Outport  Port=2  VectorParamsAs1DForOutWhenUnconnected=off
  Pos_Left_Wheel_dDispl_SteeringRod[x;y;z][] : Outport  Port=3  VectorParamsAs1DForOutWhenUnconnected=off
  w_Rel_Left_Wheel_dq_dt[qL;qR][x;y;z][rad|m] : Outport  Port=4  VectorParamsAs1DForOutWhenUnconnected=off
  w_Rel_Left_Wheel_dDispl_SteeringRod_dt[x;y;z][rad|m] : Outport  Port=5  VectorParamsAs1DForOutWhenUnconnected=off
  Pos_Right_Wheel_dq[qL;qR][x;y;z][] : Outport  Port=6  VectorParamsAs1DForOutWhenUnconnected=off
  Pos_Right_Wheel_dDispl_SteeringRod[x;y;z][] : Outport  Port=7  VectorParamsAs1DForOutWhenUnconnected=off
  w_Rel_Right_Wheel_dq_dt[qL;qR][x;y;z][rad|m] : Outport  Port=8  VectorParamsAs1DForOutWhenUnconnected=off
  w_Rel_Right_Wheel_dDispl_SteeringRod_dt[x;y;z][rad|m] : Outport  Port=9  VectorParamsAs1DForOutWhenUnconnected=off
  Pos_Left_Wheel[x;y;z][m] : Outport  Port=10  VectorParamsAs1DForOutWhenUnconnected=off
  Pos_Right_Wheel[x;y;z][m] : Outport  Port=11  VectorParamsAs1DForOutWhenUnconnected=off
  UnitVec_y_Wheel_Left[x;y;z] : Outport  Port=12  VectorParamsAs1DForOutWhenUnconnected=off
  UnitVec_y_Wheel_Right[x;y;z] : Outport  Port=13  VectorParamsAs1DForOutWhenUnconnected=off
  Displ_Spring[Left;Right][m] : Outport  Port=14  VectorParamsAs1DForOutWhenUnconnected=off
  Displ_Damper_dt[Left;Right][m|s] : Outport  Port=15  VectorParamsAs1DForOutWhenUnconnected=off
  Displ_Stabilizer[m] : Outport  Port=16  VectorParamsAs1DForOutWhenUnconnected=off
  Displ_Spring_Left_dq[qL;qR][] : Outport  Port=17  VectorParamsAs1DForOutWhenUnconnected=off
  Displ_Damper_Left_dq[qL;qR][] : Outport  Port=18  VectorParamsAs1DForOutWhenUnconnected=off
  Displ_Stabilizer_dq[qL;qR][] : Outport  Port=19  VectorParamsAs1DForOutWhenUnconnected=off
  Displ_Spring_Right_dq[qL;qR][] : Outport  Port=20  VectorParamsAs1DForOutWhenUnconnected=off
  Displ_Damper_Right_dq[qL;qR][] : Outport  Port=21  VectorParamsAs1DForOutWhenUnconnected=off
  Displ_Spring_dSteering[Left;Right][] : Outport  Port=22  VectorParamsAs1DForOutWhenUnconnected=off
  Displ_Damper_dSteering[Left;Right][] : Outport  Port=23  VectorParamsAs1DForOutWhenUnconnected=off
  Displ_Stabilizer_dSteering[Left;Right][] : Outport  Port=24  VectorParamsAs1DForOutWhenUnconnected=off
  wires:
  SUSKIN_SYM_FRONT/24 -> Displ_Stabilizer_dSteering[Left;Right][]/1
  SUSKIN_SYM_FRONT/23 -> Displ_Damper_dSteering[Left;Right][]/1
  SUSKIN_SYM_FRONT/22 -> Displ_Spring_dSteering[Left;Right][]/1
  Displ_SteeringRod_dt[Left;Right][m|s]/1 -> Terminator/1
  SUSKIN_SYM_FRONT/21 -> Displ_Damper_Right_dq[qL;qR][]/1
  SUSKIN_SYM_FRONT/20 -> Displ_Spring_Right_dq[qL;qR][]/1
  SUSKIN_SYM_FRONT/19 -> Displ_Stabilizer_dq[qL;qR][]/1
  SUSKIN_SYM_FRONT/18 -> Displ_Damper_Left_dq[qL;qR][]/1
  SUSKIN_SYM_FRONT/17 -> Displ_Spring_Left_dq[qL;qR][]/1
  SUSKIN_SYM_FRONT/16 -> Displ_Stabilizer[m]/1
  SUSKIN_SYM_FRONT/15 -> Displ_Damper_dt[Left;Right][m|s]/1
  SUSKIN_SYM_FRONT/14 -> Displ_Spring[Left;Right][m]/1
  SUSKIN_SYM_FRONT/13 -> UnitVec_y_Wheel_Right[x;y;z]/1
  SUSKIN_SYM_FRONT/12 -> UnitVec_y_Wheel_Left[x;y;z]/1
  SUSKIN_SYM_FRONT/11 -> Pos_Right_Wheel[x;y;z][m]/1
  SUSKIN_SYM_FRONT/10 -> Pos_Left_Wheel[x;y;z][m]/1
  SUSKIN_SYM_FRONT/9 -> w_Rel_Right_Wheel_dDispl_SteeringRod_dt[x;y;z][rad|m]/1
  SUSKIN_SYM_FRONT/8 -> w_Rel_Right_Wheel_dq_dt[qL;qR][x;y;z][rad|m]/1
  SUSKIN_SYM_FRONT/7 -> Pos_Right_Wheel_dDispl_SteeringRod[x;y;z][]/1
  SUSKIN_SYM_FRONT/6 -> Pos_Right_Wheel_dq[qL;qR][x;y;z][]/1
  SUSKIN_SYM_FRONT/4 -> w_Rel_Left_Wheel_dq_dt[qL;qR][x;y;z][rad|m]/1
  SUSKIN_SYM_FRONT/3 -> Pos_Left_Wheel_dDispl_SteeringRod[x;y;z][]/1
  SUSKIN_SYM_FRONT/2 -> Pos_Left_Wheel_dq[qL;qR][x;y;z][]/1
  SUSKIN_SYM_FRONT/1 -> ASMSignalBus/1
  SUSKIN_SYM_FRONT/5 -> w_Rel_Left_Wheel_dDispl_SteeringRod_dt[x;y;z][rad|m]/1
  WheelPos_Offset[x;y;z][m]/1 -> SUSKIN_SYM_FRONT/4
  Sw_Rotation[1Cardan|2ToeCamberSideView]/1 -> SUSKIN_SYM_FRONT/5
  Displ_z_dt_Wheel[Left;Right][m|s]/1 -> SUSKIN_SYM_FRONT/3
  Displ_z_Wheel[Left;Right][m]/1 -> SUSKIN_SYM_FRONT/2
  Displ_SteeringRod[Left;Right][m]/1 -> SUSKIN_SYM_FRONT/1

== system ASM_Traffic_MultiCore/VehicleDynamics/Plant/VehicleDynamics/Suspension/SuspensionRear/ASMSignalCollector ==
  BusCreator1 : BusCreator  Inputs=4
  Terminator_1 : Terminator
  Terminator_2 : Terminator
  SuspensionRear : Outport  VectorParamsAs1DForOutWhenUnconnected=off
  wires:
  BusCreator1/1 -> SuspensionRear/1  "SuspensionRear"
  [ASMBUS_SuspensionKinematicsRear] -> BusCreator1/1  "SuspensionKinematicsRear"
  [ASMBUS_SuspensionRelativeVelocitiesRear] -> Terminator_1/1
  [ASMBUS_SuspensionForceKinematicsRear] -> Terminator_2/1
  [ASMBUS_SuspensionComplianceRear] -> BusCreator1/2
  [ASMBUS_SuspensionRelativePositionRear] -> BusCreator1/4
  [ASMBUS_SuspensionForcesRear] -> BusCreator1/3

== system ASM_Traffic_MultiCore/VehicleDynamics/Plant/VehicleDynamics/Suspension/SuspensionRear/SusKin_Rear ==
  Displ_SteeringRod[Left;Right][m] : Inport
  Displ_SteeringRod_dt[Left;Right][m|s] : Inport  Port=2
  Displ_z_Wheel[Left;Right][m] : Inport  Port=3
  Displ_z_dt_Wheel[Left;Right][m|s] : Inport  Port=4
  WheelPos_Offset[x;y;z][m] : Inport  Port=5
  Sw_Rotation[1Cardan|2ToeCamberSideView] : Inport  Port=6
  SUSKIN_SYM_REAR : ASM_VehicleDynamics_lib/VehicleDynamics/Suspension/Base/SUSKIN_SYM  Tag=ASM_SUBCOMPONENT  Const_Pos_LeftWheel=MDL.VehicleDynamics.Suspension.Symmetric.Rear.Const_Pos_LeftWheel  Map_Displ_x_LeftWheel_q1q2=MDL.VehicleDynamics.Suspension.Symmetric.Rear.Map_Displ_x_LeftWheel_q1q2  Map_Displ_x_LeftWheel_q3=MDL.VehicleDynamics.Suspension.Symmetric.Rear.Map_Displ_x_LeftWheel_q3  Map_Displ_y_LeftWheel_q1q2=MDL.VehicleDynamics.Suspension.Symmetric.Rear.Map_Displ_y_LeftWheel_q1q2  Map_Displ_y_LeftWheel_q3=MDL.VehicleDynamics.Suspension.Symmetric.Rear.Map_Displ_y_LeftWheel_q3  Map_Angle_Alpha_LeftWheel_q1q2=MDL.VehicleDynamics.Suspension.Symmetric.Rear.Map_Angle_AlphaCamber_LeftWheel_q1q2  Map_Angle_Alpha_LeftWheel_q3=MDL.VehicleDynamics.Suspension.Symmetric.Rear.Map_Angle_AlphaCamber_LeftWheel_q3  Map_Angle_Beta_LeftWheel_q1q2=MDL.VehicleDynamics.Suspension.Symmetric.Rear.Map_Angle_BetaSideView_LeftWheel_q1q2  Map_Angle_Beta_LeftWheel_q3=MDL.VehicleDynamics.Suspension.Symmetric.Rear.Map_Angle_BetaSideView_LeftWheel_q3  Map_Angle_Gamma_LeftWheel_q1q2=MDL.VehicleDynamics.Suspension.Symmetric.Rear.Map_Angle_GammaToe_LeftWheel_q1q2  Map_Angle_Gamma_LeftWheel_q3=MDL.VehicleDynamics.Suspension.Symmetric.Rear.Map_Angle_GammaToe_LeftWheel_q3  Map_Displ_Spring_Left_q1q2=MDL.VehicleDynamics.Suspension.Symmetric.Rear.Map_Displ_Spring_Left_q1q2  Map_Displ_Spring_Left_q3=MDL.VehicleDynamics.Suspension.Symmetric.Rear.Map_Displ_Spring_Left_q3  Map_Displ_Damper_Left_q1q2=MDL.VehicleDynamics.Suspension.Symmetric.Rear.Map_Displ_Damper_Left_q1q2  Map_Displ_Damper_Left_q3=MDL.VehicleDynamics.Suspension.Symmetric.Rear.Map_Displ_Damper_Left_q3  Map_Displ_Stabi_Left_q1q2=MDL.VehicleDynamics.Suspension.Symmetric.Rear.Map_Displ_Stabilizer_Left_q1q2  Map_Displ_Stabi_Left_q3=MDL.VehicleDynamics.Suspension.Symmetric.Rear.Map_Displ_Stabilizer_Left_q3  ASMProperties=struct('Name','SUSKIN_SYM','Version','2.0','Library','ASM_VehicleDynamics_lib')  ASMInstanceName=suskin_sym_rear  ASMInstanceID=2
      settings: AttributesFormatString=Instance Name: %<ASMInstanceName>\nInstance ID: %<ASMInstanceID>
  Terminator : Terminator
  ASMSignalBus : Outport  VectorParamsAs1DForOutWhenUnconnected=off
  Pos_Left_Wheel_dq[qL;qR][x;y;z][] : Outport  Port=2  VectorParamsAs1DForOutWhenUnconnected=off
  Pos_Left_Wheel_dDispl_SteeringRod[x;y;z][] : Outport  Port=3  VectorParamsAs1DForOutWhenUnconnected=off
  w_Rel_Left_Wheel_dq_dt[qL;qR][x;y;z][rad|m] : Outport  Port=4  VectorParamsAs1DForOutWhenUnconnected=off
  w_Rel_Left_Wheel_dDispl_SteeringRod_dt[x;y;z][rad|m] : Outport  Port=5  VectorParamsAs1DForOutWhenUnconnected=off
  Pos_Right_Wheel_dq[qL;qR][x;y;z][] : Outport  Port=6  VectorParamsAs1DForOutWhenUnconnected=off
  Pos_Right_Wheel_dDispl_SteeringRod[x;y;z][] : Outport  Port=7  VectorParamsAs1DForOutWhenUnconnected=off
  w_Rel_Right_Wheel_dq_dt[qL;qR][x;y;z][rad|m] : Outport  Port=8  VectorParamsAs1DForOutWhenUnconnected=off
  w_Rel_Right_Wheel_dDispl_SteeringRod_dt[x;y;z][rad|m] : Outport  Port=9  VectorParamsAs1DForOutWhenUnconnected=off
  Pos_Left_Wheel[x;y;z][m] : Outport  Port=10  VectorParamsAs1DForOutWhenUnconnected=off
  Pos_Right_Wheel[x;y;z][m] : Outport  Port=11  VectorParamsAs1DForOutWhenUnconnected=off
  UnitVec_y_Wheel_Left[x;y;z] : Outport  Port=12  VectorParamsAs1DForOutWhenUnconnected=off
  UnitVec_y_Wheel_Right[x;y;z] : Outport  Port=13  VectorParamsAs1DForOutWhenUnconnected=off
  Displ_Spring[Left;Right][m] : Outport  Port=14  VectorParamsAs1DForOutWhenUnconnected=off
  Displ_Damper_dt[Left;Right][m|s] : Outport  Port=15  VectorParamsAs1DForOutWhenUnconnected=off
  Displ_Stabilizer[m] : Outport  Port=16  VectorParamsAs1DForOutWhenUnconnected=off
  Displ_Spring_Left_dq[qL;qR][] : Outport  Port=17  VectorParamsAs1DForOutWhenUnconnected=off
  Displ_Damper_Left_dq[qL;qR][] : Outport  Port=18  VectorParamsAs1DForOutWhenUnconnected=off
  Displ_Stabilizer_dq[qL;qR][] : Outport  Port=19  VectorParamsAs1DForOutWhenUnconnected=off
  Displ_Spring_Right_dq[qL;qR][] : Outport  Port=20  VectorParamsAs1DForOutWhenUnconnected=off
  Displ_Damper_Right_dq[qL;qR][] : Outport  Port=21  VectorParamsAs1DForOutWhenUnconnected=off
  Displ_Spring_dSteering[Left;Right][] : Outport  Port=22  VectorParamsAs1DForOutWhenUnconnected=off
  Displ_Damper_dSteering[Left;Right][] : Outport  Port=23  VectorParamsAs1DForOutWhenUnconnected=off
  Displ_Stabilizer_dSteering[Left;Right][] : Outport  Port=24  VectorParamsAs1DForOutWhenUnconnected=off
  wires:
  SUSKIN_SYM_REAR/24 -> Displ_Stabilizer_dSteering[Left;Right][]/1
  SUSKIN_SYM_REAR/23 -> Displ_Damper_dSteering[Left;Right][]/1
  SUSKIN_SYM_REAR/22 -> Displ_Spring_dSteering[Left;Right][]/1
  Displ_SteeringRod_dt[Left;Right][m|s]/1 -> Terminator/1
  SUSKIN_SYM_REAR/21 -> Displ_Damper_Right_dq[qL;qR][]/1
  SUSKIN_SYM_REAR/20 -> Displ_Spring_Right_dq[qL;qR][]/1
  SUSKIN_SYM_REAR/19 -> Displ_Stabilizer_dq[qL;qR][]/1
  SUSKIN_SYM_REAR/18 -> Displ_Damper_Left_dq[qL;qR][]/1
  SUSKIN_SYM_REAR/17 -> Displ_Spring_Left_dq[qL;qR][]/1
  SUSKIN_SYM_REAR/16 -> Displ_Stabilizer[m]/1
  SUSKIN_SYM_REAR/15 -> Displ_Damper_dt[Left;Right][m|s]/1
  SUSKIN_SYM_REAR/14 -> Displ_Spring[Left;Right][m]/1
  SUSKIN_SYM_REAR/13 -> UnitVec_y_Wheel_Right[x;y;z]/1
  SUSKIN_SYM_REAR/12 -> UnitVec_y_Wheel_Left[x;y;z]/1
  SUSKIN_SYM_REAR/11 -> Pos_Right_Wheel[x;y;z][m]/1
  SUSKIN_SYM_REAR/10 -> Pos_Left_Wheel[x;y;z][m]/1
  SUSKIN_SYM_REAR/9 -> w_Rel_Right_Wheel_dDispl_SteeringRod_dt[x;y;z][rad|m]/1
  SUSKIN_SYM_REAR/8 -> w_Rel_Right_Wheel_dq_dt[qL;qR][x;y;z][rad|m]/1
  SUSKIN_SYM_REAR/7 -> Pos_Right_Wheel_dDispl_SteeringRod[x;y;z][]/1
  SUSKIN_SYM_REAR/6 -> Pos_Right_Wheel_dq[qL;qR][x;y;z][]/1
  SUSKIN_SYM_REAR/4 -> w_Rel_Left_Wheel_dq_dt[qL;qR][x;y;z][rad|m]/1
  SUSKIN_SYM_REAR/3 -> Pos_Left_Wheel_dDispl_SteeringRod[x;y;z][]/1
  SUSKIN_SYM_REAR/2 -> Pos_Left_Wheel_dq[qL;qR][x;y;z][]/1
  SUSKIN_SYM_REAR/1 -> ASMSignalBus/1
  SUSKIN_SYM_REAR/5 -> w_Rel_Left_Wheel_dDispl_SteeringRod_dt[x;y;z][rad|m]/1
  WheelPos_Offset[x;y;z][m]/1 -> SUSKIN_SYM_REAR/4
  Sw_Rotation[1Cardan|2ToeCamberSideView]/1 -> SUSKIN_SYM_REAR/5
  Displ_z_dt_Wheel[Left;Right][m|s]/1 -> SUSKIN_SYM_REAR/3
  Displ_z_Wheel[Left;Right][m]/1 -> SUSKIN_SYM_REAR/2
  Displ_SteeringRod[Left;Right][m]/1 -> SUSKIN_SYM_REAR/1

== system ASM_Traffic_MultiCore/VehicleDynamics/Plant/VehicleDynamics/Tire/Tire_FL/Tire_FL ==
  Sw_Tire_Parameter_Set[1|2|3|4] : Inport
  Coeff_Fric_Road[] : Inport  Port=2
  omega_Wheel[rad|s] : Inport  Port=3
  r_Tire[m] : Inport  Port=4
  v_x_Wheel_CoorSys_CP[m|s] : Inport  Port=5
  v_y_Wheel_CoorSys_CP[m|s] : Inport  Port=6
  w_z_Wheel_CoorSys_CP[rad|s] : Inport  Port=7
  Sin_Angle_Alpha_Tire[] : Inport  Port=8
  Reset[] : Inport  Port=9
  Sw_r_Tire[1Int|2Ext] : Inport  Port=10
  r_Tire_External[m] : Inport  Port=11
  Mode[1Normal;2Mirror;3Symmetric] : Inport  Port=12
  p[Pa] : Inport  Port=13
  TIRE_TMEASY_FL : ASM_VehicleDynamics_lib/VehicleDynamics/Tire/Base/TIRE_TMEASY  Tag=ASM_SUBCOMPONENT  Para_Set_1=MDL.VehicleDynamics.Tire.FL.TME.Para_Set_1  Para_Set_2=MDL.VehicleDynamics.Tire.FL.TME.Para_Set_2  Para_Set_3=MDL.VehicleDynamics.Tire.FL.TME.Para_Set_3  Para_Set_4=MDL.VehicleDynamics.Tire.FL.TME.Para_Set_4  StepSize=SIM.StepSize  ASMProperties=struct('Name','TIRE_TMEASY','Version','2.0','Library','ASM_VehicleDynamics_lib')  ASMInstanceName=tire_tmeasy_fl  ASMInstanceID=1
      settings: AttributesFormatString=Instance Name: %<ASMInstanceName>\nInstance ID: %<ASMInstanceID>
  Terminator : Terminator
  Terminator1 : Terminator
  ASMSignalBus : Outport
  F_x_Dyn_Tire_CoorSys_CP[N] : Outport  Port=2
  F_y_Dyn_Tire_CoorSys_CP[N] : Outport  Port=3
  F_z_Dyn_Tire_CoorSys_CP[N] : Outport  Port=4
  Trq_x_CoorSys_CP[Nm] : Outport  Port=5
  Trq_y_CoorSys_W[Nm] : Outport  Port=6
  Trq_z_CoorSys_CP[Nm] : Outport  Port=7
  Stiffness_z_Tire[N|m] : Outport  Port=8
  wires:
  p[Pa]/1 -> Terminator1/1
  Mode[1Normal;2Mirror;3Symmetric]/1 -> Terminator/1
  TIRE_TMEASY_FL/5 -> Trq_x_CoorSys_CP[Nm]/1
  TIRE_TMEASY_FL/3 -> F_y_Dyn_Tire_CoorSys_CP[N]/1
  TIRE_TMEASY_FL/4 -> F_z_Dyn_Tire_CoorSys_CP[N]/1
  TIRE_TMEASY_FL/8 -> Stiffness_z_Tire[N|m]/1
  TIRE_TMEASY_FL/7 -> Trq_z_CoorSys_CP[Nm]/1
  v_x_Wheel_CoorSys_CP[m|s]/1 -> TIRE_TMEASY_FL/5
  r_Tire[m]/1 -> TIRE_TMEASY_FL/4
  r_Tire_External[m]/1 -> TIRE_TMEASY_FL/11
  Coeff_Fric_Road[]/1 -> TIRE_TMEASY_FL/2
  Reset[]/1 -> TIRE_TMEASY_FL/9
  Sin_Angle_Alpha_Tire[]/1 -> TIRE_TMEASY_FL/8
  w_z_Wheel_CoorSys_CP[rad|s]/1 -> TIRE_TMEASY_FL/7
  Sw_Tire_Parameter_Set[1|2|3|4]/1 -> TIRE_TMEASY_FL/1
  Sw_r_Tire[1Int|2Ext]/1 -> TIRE_TMEASY_FL/10
  omega_Wheel[rad|s]/1 -> TIRE_TMEASY_FL/3
  TIRE_TMEASY_FL/1 -> ASMSignalBus/1  "Tire"
  v_y_Wheel_CoorSys_CP[m|s]/1 -> TIRE_TMEASY_FL/6
  TIRE_TMEASY_FL/2 -> F_x_Dyn_Tire_CoorSys_CP[N]/1
  TIRE_TMEASY_FL/6 -> Trq_y_CoorSys_W[Nm]/1

== system ASM_Traffic_MultiCore/VehicleDynamics/Plant/VehicleDynamics/Tire/Tire_FR/Tire_FR ==
  Sw_Tire_Parameter_Set[1|2|3|4] : Inport
  Coeff_Fric_Road[] : Inport  Port=2
  omega_Wheel[rad|s] : Inport  Port=3
  r_Tire[m] : Inport  Port=4
  v_x_Wheel_CoorSys_CP[m|s] : Inport  Port=5
  v_y_Wheel_CoorSys_CP[m|s] : Inport  Port=6
  w_z_Wheel_CoorSys_CP[rad|s] : Inport  Port=7
  Sin_Angle_Alpha_Tire[] : Inport  Port=8
  Reset[] : Inport  Port=9
  Sw_r_Tire[1Int|2Ext] : Inport  Port=10
  r_Tire_External[m] : Inport  Port=11
  Mode[1Normal;2Mirror;3Symmetric] : Inport  Port=12
  p[Pa] : Inport  Port=13
  TIRE_TMEASY_FR : ASM_VehicleDynamics_lib/VehicleDynamics/Tire/Base/TIRE_TMEASY  Tag=ASM_SUBCOMPONENT  Para_Set_1=MDL.VehicleDynamics.Tire.FR.TME.Para_Set_1  Para_Set_2=MDL.VehicleDynamics.Tire.FR.TME.Para_Set_2  Para_Set_3=MDL.VehicleDynamics.Tire.FR.TME.Para_Set_3  Para_Set_4=MDL.VehicleDynamics.Tire.FR.TME.Para_Set_4  StepSize=SIM.StepSize  ASMProperties=struct('Name','TIRE_TMEASY','Version','2.0','Library','ASM_VehicleDynamics_lib')  ASMInstanceName=tire_tmeasy_fr  ASMInstanceID=2
      settings: AttributesFormatString=Instance Name: %<ASMInstanceName>\nInstance ID: %<ASMInstanceID>
  Terminator : Terminator
  Terminator1 : Terminator
  ASMSignalBus : Outport
  F_x_Dyn_Tire_CoorSys_CP[N] : Outport  Port=2
  F_y_Dyn_Tire_CoorSys_CP[N] : Outport  Port=3
  F_z_Dyn_Tire_CoorSys_CP[N] : Outport  Port=4
  Trq_x_CoorSys_CP[Nm] : Outport  Port=5
  Trq_y_CoorSys_W[Nm] : Outport  Port=6
  Trq_z_CoorSys_CP[Nm] : Outport  Port=7
  Stiffness_z_Tire[N|m] : Outport  Port=8
  wires:
  p[Pa]/1 -> Terminator1/1
  Mode[1Normal;2Mirror;3Symmetric]/1 -> Terminator/1
  TIRE_TMEASY_FR/5 -> Trq_x_CoorSys_CP[Nm]/1
  TIRE_TMEASY_FR/3 -> F_y_Dyn_Tire_CoorSys_CP[N]/1
  TIRE_TMEASY_FR/4 -> F_z_Dyn_Tire_CoorSys_CP[N]/1
  TIRE_TMEASY_FR/8 -> Stiffness_z_Tire[N|m]/1
  TIRE_TMEASY_FR/7 -> Trq_z_CoorSys_CP[Nm]/1
  v_x_Wheel_CoorSys_CP[m|s]/1 -> TIRE_TMEASY_FR/5
  r_Tire[m]/1 -> TIRE_TMEASY_FR/4
  r_Tire_External[m]/1 -> TIRE_TMEASY_FR/11
  Coeff_Fric_Road[]/1 -> TIRE_TMEASY_FR/2
  Reset[]/1 -> TIRE_TMEASY_FR/9
  Sin_Angle_Alpha_Tire[]/1 -> TIRE_TMEASY_FR/8
  w_z_Wheel_CoorSys_CP[rad|s]/1 -> TIRE_TMEASY_FR/7
  Sw_Tire_Parameter_Set[1|2|3|4]/1 -> TIRE_TMEASY_FR/1
  Sw_r_Tire[1Int|2Ext]/1 -> TIRE_TMEASY_FR/10
  omega_Wheel[rad|s]/1 -> TIRE_TMEASY_FR/3
  TIRE_TMEASY_FR/1 -> ASMSignalBus/1  "Tire"
  v_y_Wheel_CoorSys_CP[m|s]/1 -> TIRE_TMEASY_FR/6
  TIRE_TMEASY_FR/2 -> F_x_Dyn_Tire_CoorSys_CP[N]/1
  TIRE_TMEASY_FR/6 -> Trq_y_CoorSys_W[Nm]/1
